simulink model "Mapping_cs"  (R2019a)
settings: Solver=ode5  StartTime=0.0  StopTime=inf  FixedStep=1/20  RelTol=1e-3
PreLoadFcn:
  | mbxruntime.callbacks.PreLoadFcn(bdroot);
PostLoadFcn:
  | mbxruntime.callbacks.PostLoadFcn(bdroot);
InitFcn:
  | mbxruntime.callbacks.InitFcn(bdroot);
StartFcn:
  | mbxruntime.callbacks.StartFcn(bdroot);
StopFcn:
  | mbxruntime.callbacks.StopFcn(bdroot);
model workspace: external: MAT-File .\Mapping_cs_hws.mat (data not in the file)
undefined symbols (not defined in the file or in its folder): InitImageOutputDir, Mapping_cs_BMW_X5_SUV_1_Path_pathUniqueID, Mapping_cs_BMW_X5_SUV_1_SpeedProfile_speedProfileUniqueID, mbxruntime
libraries: PreScanUsefulBlocks x1, adeye_lib x1
(part 1 of 2)
CloseFcn:
  | mbxruntime.callbacks.CloseFcn(bdroot);
settings Model: Creator=PRESCAN  LastModifiedBy=adeye
settings DataIOCC: LimitDataPoints=on  SaveFormat=Array  SignalLoggingSaveFormat=ModelDataLogs  ReturnWorkspaceOutputs=off
settings OptimizationCC: DefaultParameterBehavior=Inlined  ExpressionDepthLimit=2147483647  InitFltsAndDblsToZero=on  LifeSpan=inf
settings DebuggingCC: SaveWithParameterizedLinksMsg=none  UnderspecifiedInitializationDetection=Classic  MergeDetectMultiDrivingBlocksExec=none  SignalResolutionControl=TryResolveAllWithWarning  MultiTaskDSMMsg=warning  MultiTaskCondExecSysMsg=none  FcnCallInpInsideContextMsg=warning  StateNameClashWarn=warning  SFUnexpectedBacktrackingDiag=warning  SFNoUnconditionalDefaultTransitionDiag=warning  SFExecutionAtInitializationDiag=none  ArithmeticOperatorsInVariantConditions=warning
settings HardwareCC: ProdBitPerPointer=32  ProdBitPerSizeT=32  ProdBitPerPtrDiffT=32  ProdLargestAtomicFloat=None  ProdIntDivRoundTo=Undefined  ProdEndianess=Unspecified  ProdWordSize=32  ProdHWDeviceType=32-bit Generic
settings ModelReferenceCC: UpdateModelReferenceTargets=IfOutOfDate  PropagateSignalLabelsOutOfModel=off
settings SFSimCC: SimUseLocalCustomCode=off  SimParseCustomCode=off
settings SFSimCC: SimCustomHeaderCode=|
  | #include "prescan.h"
  | #include "prescan_platform.h"
  | #include "prescan_aimsunturnindicatorsetter_data.h"
settings RTWCC: RTWUseLocalCustomCode=off
settings CodeAppCC: StateflowObjectComments=on
settings GRTTargetCC: TargetFcnLib=ansi_tfl_tmw.mat  TargetLangStandard=C89/C90 (ANSI)  GeneratePreprocessorConditionals=Disable all  CombineOutputUpdateFcns=off  GRTInterface=on
settings ConfigComp: CovMetricSettings=dw  CovHtmlReporting=on  CovSaveCumulativeToWorkspaceVar=on  CovSaveSingleToWorkspaceVar=on  CovExternalEMLEnable=off  CovSFcnEnable=off

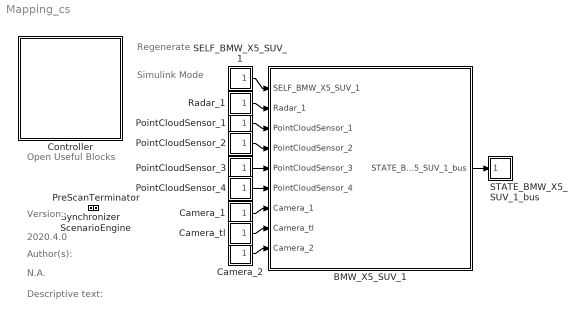
== system Mapping_cs ==
  note: Regenerate
  note: Simulink Mode
  note: Open Useful Blocks
  note: 2020.4.0
  note: Version:
  note: Author(s):
  note: N.A.
  note: Descriptive text:
  BMW_X5_SUV_1 : Subsystem  Tag=WorldObjectSubSystem  InitFcn=UniqueId = '158';
      mask init:
      | modelPath = GenericModelHelper.getGenericModelFilePath('ModelDepo','Vehicles\BMW_X5\BMW_X5.pgmb','bfeb1c11467705ab888b3011684c848b');imagePath = GenericModelHelper.getCompilationPicture(modelPath, 'BMW_X5_HighPoly.png');
      mask Display: image(imread(imagePath));color('white');text(0, 0, ' ID=10\n')
  Camera_1 : Subsystem  Tag=sensor/Camera/CameraSensor  Priority=30  mask(PreScan Source Block: Camera Sensor){}
      mask help: The Camera Sensor provides a color or monochrome image.
      settings: OpenFcn=open_system([gcb '/Sensor'],'mask')
      mask Help: eval('openHelp(457)')
      mask Display: image(imread('CameraSensor.png'))
  Camera_2 : Subsystem  Tag=sensor/Camera/CameraSensor  Priority=30  mask(PreScan Source Block: Camera Sensor){}
      mask help: The Camera Sensor provides a color or monochrome image.
      settings: OpenFcn=open_system([gcb '/Sensor'],'mask')
      mask Help: eval('openHelp(457)')
      mask Display: image(imread('CameraSensor.png'))
  Camera_tl : Subsystem  Tag=sensor/Camera/CameraSensor  Priority=30  mask(PreScan Source Block: Camera Sensor){}
      mask help: The Camera Sensor provides a color or monochrome image.
      settings: OpenFcn=open_system([gcb '/Sensor'],'mask')
      mask Help: eval('openHelp(457)')
      mask Display: image(imread('CameraSensor.png'))
  Controller : Subsystem  Description=8A3CD2955739A82C886C20AE3E253D78460D53180EE2C1B14CC08DF75A70BE77  Priority=-1  LoadFcn=load PreScanControllerData  mask(PreScan Simulation Controller){prescanversion='2020.4.0', ModelReferencing=off, TimeStep=1/20, ControlMode=0, PreScanExecutionMode=on, ControllerCount=0, ControllerIndex=0, ControllerOptions=''}
      mask prompts: prescanversion "PreScan Version"; ModelReferencing "Use Model Referencing"; TimeStep "Upload Period [s]"; ControlMode "Control Mode"; PreScanExecutionMode "Execution Mode"; ControllerCount "Controller Count"; ControllerIndex "Controller Index"; ControllerOptions "Controller Options"
      mask help:
      | Please do not remove this block from the compilation sheet,
      | as it connects the model to the PreScan environment.
      mask init:
      | model = bdroot(gcb);
      | ExperimentFile = mbxruntime.findExperimentFile(model,true); %relative path
      | 
      | [d1, d2, d3, prescandata] = prescan_Settings();
      | ModelDepo = fullfile(prescandata,'ModelDepo'); 
      | 
      | RTmode = mbxruntime.getRTMode(model);
      | 
      | SimulationMode = get_param(bdroot,'SimulationMode');
      | if strcmp(SimulationMode, 'rapid-accelerator')
      |     SimulationMode = 'external';
      | end
      | TargetName = get_param(bdroot,'SystemTargetFile');
      settings: ModelCloseFcn=assignin('base',['model_closed_' bdroot],true);
      mask Help: eval('openHelp(812)')
      mask Display: image(imread('prescanlogo.ico'))
  PointCloudSensor_1 : Subsystem  Tag=sensor/PointCloudInport  Priority=30  mask(PreScan Source Block: Point Cloud Sensor){}
      mask help: The Point Cloud Sensor provides XYZ positions relative to the sensor
      settings: OpenFcn=open_system([gcb '/Sensor'],'mask')
      mask Help: eval('openHelp(6400)')
      mask Display: image(imread('PointCloudSensorSL.png'))
  PointCloudSensor_2 : Subsystem  Tag=sensor/PointCloudInport  Priority=30  mask(PreScan Source Block: Point Cloud Sensor){}
      mask help: The Point Cloud Sensor provides XYZ positions relative to the sensor
      settings: OpenFcn=open_system([gcb '/Sensor'],'mask')
      mask Help: eval('openHelp(6400)')
      mask Display: image(imread('PointCloudSensorSL.png'))
  PointCloudSensor_3 : Subsystem  Tag=sensor/PointCloudInport  Priority=30  mask(PreScan Source Block: Point Cloud Sensor){}
      mask help: The Point Cloud Sensor provides XYZ positions relative to the sensor
      settings: OpenFcn=open_system([gcb '/Sensor'],'mask')
      mask Help: eval('openHelp(6400)')
      mask Display: image(imread('PointCloudSensorSL.png'))
  PointCloudSensor_4 : Subsystem  Tag=sensor/PointCloudInport  Priority=30  mask(PreScan Source Block: Point Cloud Sensor){}
      mask help: The Point Cloud Sensor provides XYZ positions relative to the sensor
      settings: OpenFcn=open_system([gcb '/Sensor'],'mask')
      mask Help: eval('openHelp(6400)')
      mask Display: image(imread('PointCloudSensorSL.png'))
  PreScanTerminator : Subsystem  Tag=PreScanTerminator  Priority=999  LoadFcn=load PrescanTerminatorData  mask(PreScan Simulation Terminator){TimeStep=1/20}
      mask prompts: TimeStep "Upload Period [s]"
      mask help:
      | Please do not remove this block from the compilation sheet as it
      | connects the model to the PreScan environment.
      mask Help: eval('openHelp(812)')
      mask Display: image(imread('prescanlogo.ico'))
  Radar_1 : Subsystem  Tag=sensor/Radar  Priority=30  LoadFcn=load('PrescanScannerSensorData.mat');load('PrescanScannerSensorMessage.mat')  mask(PreScan Source Block: Radar Sensor){}
      mask help:
      | The Radar Sensor is a detailed sensor based on a physical radar
      | model that includes Antenna GAIN Maps (AGM) and atmospheric
      | attenuation.
      |
      | For more information, please click Help.
      settings: OpenFcn=open_system([gcb '/Sensor'],'mask')
      mask Help: eval('openHelp(1464)')
      mask Display: image(imread('Radar.png'))
  SELF_BMW_X5_SUV_1 : Subsystem  Tag=sensor/SelfPort  Priority=30  LoadFcn=load('PreScanSelfSensorData.mat')  mask(PreScan Source Block: SELF){}
      mask help:
      | The SELF port shows (state) information of the actor itself. The outputs are position in the experiment's axis system and the GPS coordinates, and the object's absolute velocity and compass heading.
      |
      | For more information, please click Help.
      settings: OpenFcn=open_system([gcb '/Sensor'],'mask')
      mask Help: eval('openHelp(462)')
      mask Display: image(imread('GPS.png'))
  STATE_BMW_X5_SUV_1_bus : Subsystem  Tag=actuator/StatePort  Priority=0  LoadFcn=load('PreScanStateActuatorData.mat')  mask(PreScan Sink Block: State){}
      mask help:
      | The Actor State contains a vector signal of size (9x1), containing the following signals:
      |
      | -  Position    	(x,y,z)             	[m]
      | -  Velocity    	(vx,vy,vz)         	[m/s]
      | -  Angles       	(Roll, Pitch, Yaw)	[rad]
      |
      | The Actor state is defined in the global axis system.
      | The state is superponed on the Initial position defined in the GUI.
      |
      | For more information, please click Help.
      settings: OpenFcn=open_system([gcb '/Actuator'],'mask')
      mask Help: eval('openHelp(222)')
      mask Display: image(imread('State.png'))
  ScenarioEngine : Subsystem  Tag=PreScanOpenScenarioBlock  Priority=10  LoadFcn=load PrescanSynchronizeData  mask(PreScan Simulation Core Block){TimeStep=1/20}
      mask prompts: TimeStep "Timestep [s]"
      mask help:
      | Please do not remove this block from the PreScan compilation sheet,
      | as it contains essential configuration parameters for a PreScan simulation.
      settings: DeleteFcn=PreScanBlockDeleteFcn;
      mask Display: image(imread('prescanlogo.ico'))
  Synchronizer : Subsystem  Tag=PreScanSynchronizer  Priority=20  LoadFcn=load PrescanSynchronizeData  mask(PreScan Simulation Core Block){TimeStep=1/20}
      mask prompts: TimeStep "Timestep [s]"
      mask help:
      | Please do not remove this block from the PreScan compilation sheet,
      | as it contains essential configuration parameters for a PreScan simulation.
      settings: DeleteFcn=PreScanBlockDeleteFcn;
      mask Display: image(imread('prescanlogo.ico'))
  wires:
  BMW_X5_SUV_1/1(STATE_BMW_X5_SUV_1_bus) -> STATE_BMW_X5_SUV_1_bus/1(STATE_BMW_X5_SUV_1_bus)
  SELF_BMW_X5_SUV_1/1(SELF_BMW_X5_SUV_1) -> BMW_X5_SUV_1/1(SELF_BMW_X5_SUV_1)
  Radar_1/1(Radar_1) -> BMW_X5_SUV_1/2(Radar_1)
  PointCloudSensor_1/1(PointCloudSensor_1) -> BMW_X5_SUV_1/3(PointCloudSensor_1)
  PointCloudSensor_2/1(PointCloudSensor_2) -> BMW_X5_SUV_1/4(PointCloudSensor_2)
  PointCloudSensor_3/1(PointCloudSensor_3) -> BMW_X5_SUV_1/5(PointCloudSensor_3)
  PointCloudSensor_4/1(PointCloudSensor_4) -> BMW_X5_SUV_1/6(PointCloudSensor_4)
  Camera_1/1(Camera_1) -> BMW_X5_SUV_1/7(Camera_1)
  Camera_tl/1(Camera_tl) -> BMW_X5_SUV_1/8(Camera_tl)
  Camera_2/1(Camera_2) -> BMW_X5_SUV_1/9(Camera_2)

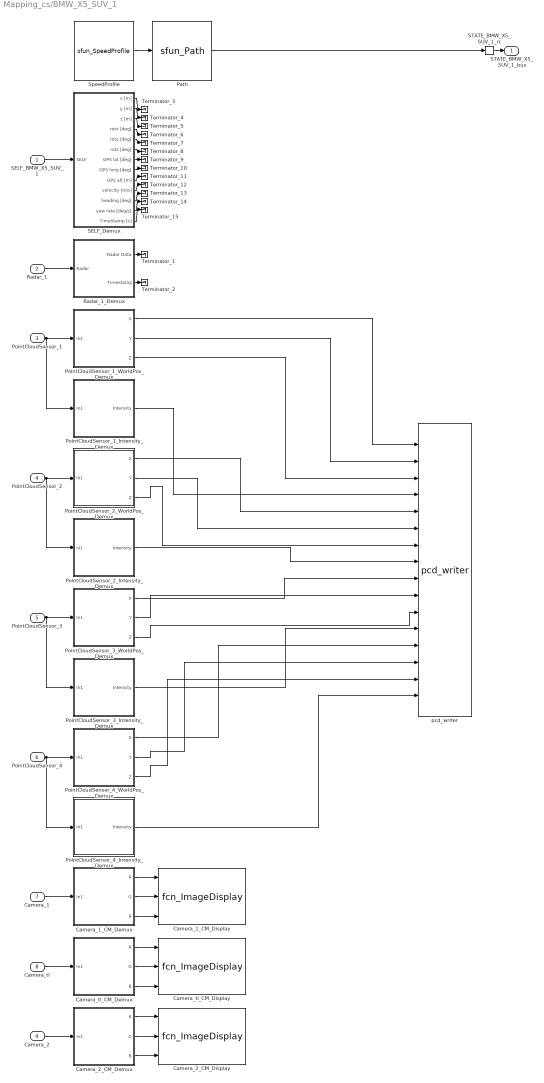
== system Mapping_cs/BMW_X5_SUV_1 ==
  SELF_BMW_X5_SUV_1 : Inport  Tag=inport/SelfPort  OutDataTypeStr=Bus: PRESCAN_SELFSENSORDATA  PortDimensions=1  SampleTime=1/20  BusOutputAsStruct=on
  Radar_1 : Inport  Tag=inport/Radar  Port=2  OutDataTypeStr=Bus: PRESCAN_SCANNERSENSOR_MESSAGE  PortDimensions=7  SampleTime=1/20  BusOutputAsStruct=on
  PointCloudSensor_1 : Inport  Tag=inport/PointCloudInport  Port=3  OutDataTypeStr=single  SampleTime=1/20  BusOutputAsStruct=on
  PointCloudSensor_2 : Inport  Tag=inport/PointCloudInport  Port=4  OutDataTypeStr=single  SampleTime=1/20  BusOutputAsStruct=on
  PointCloudSensor_3 : Inport  Tag=inport/PointCloudInport  Port=5  OutDataTypeStr=single  SampleTime=1/20  BusOutputAsStruct=on
  PointCloudSensor_4 : Inport  Tag=inport/PointCloudInport  Port=6  OutDataTypeStr=single  SampleTime=1/20  BusOutputAsStruct=on
  Camera_1 : Inport  Tag=inport/Camera/CameraSensor  Port=7  OutDataTypeStr=uint8  SampleTime=1/20  BusOutputAsStruct=on
  Camera_tl : Inport  Tag=inport/Camera/CameraSensor  Port=8  OutDataTypeStr=uint8  SampleTime=1/20  BusOutputAsStruct=on
  Camera_2 : Inport  Tag=inport/Camera/CameraSensor  Port=9  OutDataTypeStr=uint8  SampleTime=1/20  BusOutputAsStruct=on
  Camera_1_CM_Demux : Subsystem  Tag=demux/Camera/Color  mask{SensorName=Camera_1, hres=960, vres=720}
      mask prompts: SensorName "Sensor Name"; hres "Horizontal Resolution"; vres "Vertical Resolution"
      mask Help: eval('openHelp(457)')
      mask Display:
      | fprintf('MONO CAMERA:\n Color\n %s \n %d x %d px',SensorName,hres,vres)
      | port_label('output',1,'R')
      | port_label('output',2,'G')
      | port_label('output',3,'B')
  Camera_1_CM_Display : M-S-Function  Tag=CameraSensor_Color_Display  InitFcn=InitImageOutputDir(gcb);  FunctionName=fcn_ImageDisplay  Parameters=SensorName EnableDisplay EnablePosition DisplayPosition FigureHandle SaveResults BitmapFormat TempOutputDir CameraType DataType  mask(PreScan Color Display Block){SensorName=Camera_1, EnableDisplay=on, EnablePosition=off, DisplayPosition=[10 10 960 720], FigureHandle=15805, SaveResults=off, Format=PNG, TempOutputDir=0, CameraType=Mono, DataType=uint8}
      mask prompts: SensorName "User Specified: Title of Display"; EnableDisplay "Active"; EnablePosition "Set Display window position"; DisplayPosition "Display window position [xpos ypos width height]"; FigureHandle "Unique Handle"; SaveResults "Save results"; TempOutputDir "OutputDir"; CameraType "Camera Type"; DataType "Image Data Type"
      mask help: This block displays the RGB output of a PreScan camera sensor.
      mask init:
      | if EnableDisplay
      |     EnableString='';
      |     EnableColor='gray';
      | else
      |     EnableString='INACTIVE';
      |     EnableColor='red';
      | end
      | switch Format
      |     case 1
      |         BitmapFormat = 'png';
      |     case 2
      |         BitmapFormat = 'bmp';
      |     case 3
      |         BitmapFormat = 'jpg';
      | end 
      | if CameraType==1
      |     CameraTypeName='MONO';
      |     PortNumber=0;
      | else
      |     CameraTypeName='STEREO';
      |     PortNumber=3;
      | end
      settings: CopyFcn=CopyFcnDisplay  DeleteFcn=PreScanBlockDeleteFcn;  ModelCloseFcn=fcn_ImageDisplay_ModelCloseFcn
      mask Help: eval('openHelp(457)')
      mask Callback EnablePosition:
      | MV=get_param(gcb,'MaskVisibilities');
      | if strcmp(get_param(gcb,'EnablePosition'),'on')
      |     MV{4}='on';
      | else
      |     MV{4}='off';
      | end
      | set_param(gcb,'MaskVisibilities',MV);
      | clear MV;
      mask TypeOptions Format: PNG | BMP | JPG
      mask TypeOptions CameraType: Mono | Stereo
      mask TypeOptions DataType: uint8 | single
      mask Display:
      | color(EnableColor);
      | fprintf('%s\n DISPLAY:\n Color \n %s',EnableString,SensorName)
      | port_label('input',1,'R')
      | port_label('input',2,'G')
      | port_label('input',3,'B')
      | port_label('input',PortNumber+1,'R')
      | port_label('input',PortNumber+2,'G')
      | port_label('input',PortNumber+3,'B')
  Camera_2_CM_Demux : Subsystem  Tag=demux/Camera/Color  mask{SensorName=Camera_2, hres=960, vres=720}
      mask prompts: SensorName "Sensor Name"; hres "Horizontal Resolution"; vres "Vertical Resolution"
      mask Help: eval('openHelp(457)')
      mask Display:
      | fprintf('MONO CAMERA:\n Color\n %s \n %d x %d px',SensorName,hres,vres)
      | port_label('output',1,'R')
      | port_label('output',2,'G')
      | port_label('output',3,'B')
  Camera_2_CM_Display : M-S-Function  Tag=CameraSensor_Color_Display  InitFcn=InitImageOutputDir(gcb);  FunctionName=fcn_ImageDisplay  Parameters=SensorName EnableDisplay EnablePosition DisplayPosition FigureHandle SaveResults BitmapFormat TempOutputDir CameraType DataType  mask(PreScan Color Display Block){SensorName=Camera_2, EnableDisplay=on, EnablePosition=off, DisplayPosition=[10 10 960 720], FigureHandle=15807, SaveResults=off, Format=PNG, TempOutputDir=0, CameraType=Mono, DataType=uint8}
      mask prompts: SensorName "User Specified: Title of Display"; EnableDisplay "Active"; EnablePosition "Set Display window position"; DisplayPosition "Display window position [xpos ypos width height]"; FigureHandle "Unique Handle"; SaveResults "Save results"; TempOutputDir "OutputDir"; CameraType "Camera Type"; DataType "Image Data Type"
      mask help: This block displays the RGB output of a PreScan camera sensor.
      mask init: same as Mapping_cs/BMW_X5_SUV_1/Camera_1_CM_Display
      settings: CopyFcn=CopyFcnDisplay  DeleteFcn=PreScanBlockDeleteFcn;  ModelCloseFcn=fcn_ImageDisplay_ModelCloseFcn
      mask Help: eval('openHelp(457)')
      mask Callback EnablePosition:
      | MV=get_param(gcb,'MaskVisibilities');
      | if strcmp(get_param(gcb,'EnablePosition'),'on')
      |     MV{4}='on';
      | else
      |     MV{4}='off';
      | end
      | set_param(gcb,'MaskVisibilities',MV);
      | clear MV;
      mask TypeOptions Format: PNG | BMP | JPG
      mask TypeOptions CameraType: Mono | Stereo
      mask TypeOptions DataType: uint8 | single
      mask Display:
      | color(EnableColor);
      | fprintf('%s\n DISPLAY:\n Color \n %s',EnableString,SensorName)
      | port_label('input',1,'R')
      | port_label('input',2,'G')
      | port_label('input',3,'B')
      | port_label('input',PortNumber+1,'R')
      | port_label('input',PortNumber+2,'G')
      | port_label('input',PortNumber+3,'B')
  Camera_tl_CM_Demux : Subsystem  Tag=demux/Camera/Color  mask{SensorName=Camera_tl, hres=960, vres=720}
      mask prompts: SensorName "Sensor Name"; hres "Horizontal Resolution"; vres "Vertical Resolution"
      mask Help: eval('openHelp(457)')
      mask Display:
      | fprintf('MONO CAMERA:\n Color\n %s \n %d x %d px',SensorName,hres,vres)
      | port_label('output',1,'R')
      | port_label('output',2,'G')
      | port_label('output',3,'B')
  Camera_tl_CM_Display : M-S-Function  Tag=CameraSensor_Color_Display  InitFcn=InitImageOutputDir(gcb);  FunctionName=fcn_ImageDisplay  Parameters=SensorName EnableDisplay EnablePosition DisplayPosition FigureHandle SaveResults BitmapFormat TempOutputDir CameraType DataType  mask(PreScan Color Display Block){SensorName=Camera_tl, EnableDisplay=on, EnablePosition=off, DisplayPosition=[10 10 960 720], FigureHandle=15806, SaveResults=off, Format=PNG, TempOutputDir=0, CameraType=Mono, DataType=uint8}
      mask prompts: SensorName "User Specified: Title of Display"; EnableDisplay "Active"; EnablePosition "Set Display window position"; DisplayPosition "Display window position [xpos ypos width height]"; FigureHandle "Unique Handle"; SaveResults "Save results"; TempOutputDir "OutputDir"; CameraType "Camera Type"; DataType "Image Data Type"
      mask help: This block displays the RGB output of a PreScan camera sensor.
      mask init: same as Mapping_cs/BMW_X5_SUV_1/Camera_1_CM_Display
      settings: CopyFcn=CopyFcnDisplay  DeleteFcn=PreScanBlockDeleteFcn;  ModelCloseFcn=fcn_ImageDisplay_ModelCloseFcn
      mask Help: eval('openHelp(457)')
      mask Callback EnablePosition:
      | MV=get_param(gcb,'MaskVisibilities');
      | if strcmp(get_param(gcb,'EnablePosition'),'on')
      |     MV{4}='on';
      | else
      |     MV{4}='off';
      | end
      | set_param(gcb,'MaskVisibilities',MV);
      | clear MV;
      mask TypeOptions Format: PNG | BMP | JPG
      mask TypeOptions CameraType: Mono | Stereo
      mask TypeOptions DataType: uint8 | single
      mask Display:
      | color(EnableColor);
      | fprintf('%s\n DISPLAY:\n Color \n %s',EnableString,SensorName)
      | port_label('input',1,'R')
      | port_label('input',2,'G')
      | port_label('input',3,'B')
      | port_label('input',PortNumber+1,'R')
      | port_label('input',PortNumber+2,'G')
      | port_label('input',PortNumber+3,'B')
  Path : S-Function  LoadFcn=load('PrescanMotionData.mat')  FunctionName=sfun_Path  Parameters=mbxruntime.parameters.convert(uniqueID), pathUniqueID, mbxruntime.parameters.convert(timestep)  SFunctionDeploymentMode=off  EnableBusSupport=off  mask(Path){uniqueID=158, pathUniqueID=Mapping_cs_BMW_X5_SUV_1_Path_pathUniqueID, timestep=1/20}
      mask prompts: uniqueID "Object Unique ID"; pathUniqueID "Path Unique ID"; timestep "MATLAB timestep:"
      mask help:
      | The path block outputs the position along a given trajectory.
      |
      | For more information, please click Help.
      mask Help: eval('openHelp(312)')
      mask Display: image(imread('Path.png'))
  PointCloudSensor_1_Intensity_Demux : Subsystem  Tag=demux/PCS/Intensity  mask{SensorName=PointCloudSensor_1, offset=675, hres=225, vres=16}
      mask prompts: SensorName "Sensor Name"; offset "Data Start"; hres "Horizontal Resolution"; vres "Vertical Resolution"
      mask Help: eval('openHelp(6400)')
      mask Display:
      | fprintf('Point Cloud:\n Data\n %s \n %d x %d px',SensorName,hres,vres)
      | port_label('output',1,'Intensity')
  PointCloudSensor_1_WorldPos_Demux : Subsystem  Tag=demux/PCS/WorldPos  mask{SensorName=PointCloudSensor_1, offset=0, hres=225, vres=16}
      mask prompts: SensorName "Sensor Name"; offset "Data Start"; hres "Horizontal Resolution"; vres "Vertical Resolution"
      mask Help: eval('openHelp(6400)')
      mask Display:
      | fprintf('Point Cloud:\n Data\n %s \n %d x %d px',SensorName,hres,vres)
      | port_label('output',1,'X')
      | port_label('output',2,'Y')
      | port_label('output',3,'Z')
  PointCloudSensor_2_Intensity_Demux : Subsystem  Tag=demux/PCS/Intensity  mask{SensorName=PointCloudSensor_2, offset=675, hres=225, vres=16}
      mask prompts: SensorName "Sensor Name"; offset "Data Start"; hres "Horizontal Resolution"; vres "Vertical Resolution"
      mask Help: eval('openHelp(6400)')
      mask Display:
      | fprintf('Point Cloud:\n Data\n %s \n %d x %d px',SensorName,hres,vres)
      | port_label('output',1,'Intensity')
  PointCloudSensor_2_WorldPos_Demux : Subsystem  Tag=demux/PCS/WorldPos  mask{SensorName=PointCloudSensor_2, offset=0, hres=225, vres=16}
      mask prompts: SensorName "Sensor Name"; offset "Data Start"; hres "Horizontal Resolution"; vres "Vertical Resolution"
      mask Help: eval('openHelp(6400)')
      mask Display:
      | fprintf('Point Cloud:\n Data\n %s \n %d x %d px',SensorName,hres,vres)
      | port_label('output',1,'X')
      | port_label('output',2,'Y')
      | port_label('output',3,'Z')
  PointCloudSensor_3_Intensity_Demux : Subsystem  Tag=demux/PCS/Intensity  mask{SensorName=PointCloudSensor_3, offset=675, hres=225, vres=16}
      mask prompts: SensorName "Sensor Name"; offset "Data Start"; hres "Horizontal Resolution"; vres "Vertical Resolution"
      mask Help: eval('openHelp(6400)')
      mask Display:
      | fprintf('Point Cloud:\n Data\n %s \n %d x %d px',SensorName,hres,vres)
      | port_label('output',1,'Intensity')
  PointCloudSensor_3_WorldPos_Demux : Subsystem  Tag=demux/PCS/WorldPos  mask{SensorName=PointCloudSensor_3, offset=0, hres=225, vres=16}
      mask prompts: SensorName "Sensor Name"; offset "Data Start"; hres "Horizontal Resolution"; vres "Vertical Resolution"
      mask Help: eval('openHelp(6400)')
      mask Display:
      | fprintf('Point Cloud:\n Data\n %s \n %d x %d px',SensorName,hres,vres)
      | port_label('output',1,'X')
      | port_label('output',2,'Y')
      | port_label('output',3,'Z')
  PointCloudSensor_4_Intensity_Demux : Subsystem  Tag=demux/PCS/Intensity  mask{SensorName=PointCloudSensor_4, offset=675, hres=225, vres=16}
      mask prompts: SensorName "Sensor Name"; offset "Data Start"; hres "Horizontal Resolution"; vres "Vertical Resolution"
      mask Help: eval('openHelp(6400)')
      mask Display:
      | fprintf('Point Cloud:\n Data\n %s \n %d x %d px',SensorName,hres,vres)
      | port_label('output',1,'Intensity')
  PointCloudSensor_4_WorldPos_Demux : Subsystem  Tag=demux/PCS/WorldPos  mask{SensorName=PointCloudSensor_4, offset=0, hres=225, vres=16}
      mask prompts: SensorName "Sensor Name"; offset "Data Start"; hres "Horizontal Resolution"; vres "Vertical Resolution"
      mask Help: eval('openHelp(6400)')
      mask Display:
      | fprintf('Point Cloud:\n Data\n %s \n %d x %d px',SensorName,hres,vres)
      | port_label('output',1,'X')
      | port_label('output',2,'Y')
      | port_label('output',3,'Z')
  Radar_1_Demux : Subsystem  Tag=demux/Radar  TreatAsAtomicUnit=on  mask(PreScan Demux Block: Radar){MAXMESSAGES=7}
      mask prompts: MAXMESSAGES "Number of Objects"
      mask help:
      | The Radar Sensor is a detailed sensor based on a physical radar
      | model that includes Antenna GAIN Maps (AGM) and atmospheric
      | attenuation.
      |
      | For more information, please click Help.
      mask Help: eval('openHelp(1464)')
      mask Display:
      | port_label('input',1,'Radar')
      | port_label('output',1,'Radar Data')
      | port_label('output',2,'Timestamp [s]')
  SELF_Demux : Subsystem  Tag=demux/SelfPort  mask(PreScan Demux Block:){}
      mask help:
      | The SELF port shows (state) information of the actor itself. The outputs are position in the experiment's axis system and the GPS coordinates, and the object's absolute velocity and compass heading.
      |
      | For more information, please click Help.
      settings: DeleteFcn=PreScanBlockDeleteFcn;
      mask Help: eval('openHelp(462)')
      mask Display:
      | port_label('output',1,'x [m]')
      | port_label('output',2,'y [m]')
      | port_label('output',3,'z [m]','texmode','on')
      | port_label('output',4,'Rotx [deg]','texmode','on')
      | port_label('output',5,'Roty [deg]','texmode','on')
      | port_label('output',6,'Rotz [deg]','texmode','on')
      | port_label('output',7,'GPS lat [deg]','texmode','on')
      | port_label('output',8,'GPS long [deg]','texmode','on')
      | port_label('output',9,'GPS alt [m]','texmode','on')
      | port_label('output',10,'Velocity [m/s]')
      | port_label('output',11,'Heading [deg]')
      | port_label('output',12,'Yaw rate [deg/s]')
      | port_label('output',13,'Timestamp [s]')
  STATE_BMW_X5_SUV_1_rc : RateTransition  Tag=mux_rc/StatePort  OutPortSampleTimeOpt=Inherit
  SpeedProfile : S-Function  LoadFcn=load('PrescanMotionData.mat')  FunctionName=sfun_SpeedProfile  Parameters=speedProfileUniqueID, mbxruntime.parameters.convert(timestep)  SFunctionDeploymentMode=off  EnableBusSupport=off  mask(SpeedProfile){speedProfileUniqueID=Mapping_cs_BMW_X5_SUV_1_SpeedProfile_speedProfileUniqueID, timestep=1/20}
      mask prompts: speedProfileUniqueID "Speed Profile Unique ID"; timestep "MATLAB timestep:"
      mask help:
      | The speed profile block outputs the travelled distance, velocities and acceleration along a given path.
      |
      | For more information, please click Help.
      mask Help: eval('openHelp(312)')
      mask Display: image(imread('SpeedProfile.png'))
  Terminator_{1..15} (15 alike) : Terminator
  pcd_writer : adeye_lib/pcd_writer  SystemSampleTime=-1
  STATE_BMW_X5_SUV_1_bus : Outport  Tag=outport/StatePort  OutDataTypeStr=Bus: PRESCAN_STATEACTUATORDATA  PortDimensions=1  SampleTime=1/20
  wires:
  STATE_BMW_X5_SUV_1_rc/1 -> STATE_BMW_X5_SUV_1_bus/1
  SpeedProfile/1 -> Path/1
  Path/1 -> STATE_BMW_X5_SUV_1_rc/1
  SELF_BMW_X5_SUV_1/1 -> SELF_Demux/1(SELF)
  Radar_1/1 -> Radar_1_Demux/1(Radar)
  PointCloudSensor_1/1 -> PointCloudSensor_1_WorldPos_Demux/1(In1), PointCloudSensor_1_Intensity_Demux/1(In1)
  PointCloudSensor_1_WorldPos_Demux/1(X) -> pcd_writer/1
  PointCloudSensor_1_WorldPos_Demux/2(Y) -> pcd_writer/2
  PointCloudSensor_1_WorldPos_Demux/3(Z) -> pcd_writer/3
  PointCloudSensor_1_Intensity_Demux/1(Intensity) -> pcd_writer/4
  PointCloudSensor_2/1 -> PointCloudSensor_2_WorldPos_Demux/1(In1), PointCloudSensor_2_Intensity_Demux/1(In1)
  PointCloudSensor_2_WorldPos_Demux/1(X) -> pcd_writer/5
  PointCloudSensor_2_WorldPos_Demux/2(Y) -> pcd_writer/6
  PointCloudSensor_2_WorldPos_Demux/3(Z) -> pcd_writer/7
  PointCloudSensor_2_Intensity_Demux/1(Intensity) -> pcd_writer/8
  PointCloudSensor_3/1 -> PointCloudSensor_3_WorldPos_Demux/1(In1), PointCloudSensor_3_Intensity_Demux/1(In1)
  PointCloudSensor_3_WorldPos_Demux/1(X) -> pcd_writer/9
  PointCloudSensor_3_WorldPos_Demux/2(Y) -> pcd_writer/10
  PointCloudSensor_3_WorldPos_Demux/3(Z) -> pcd_writer/11
  PointCloudSensor_3_Intensity_Demux/1(Intensity) -> pcd_writer/12
  PointCloudSensor_4/1 -> PointCloudSensor_4_WorldPos_Demux/1(In1), PointCloudSensor_4_Intensity_Demux/1(In1)
  PointCloudSensor_4_WorldPos_Demux/1(X) -> pcd_writer/13
  PointCloudSensor_4_WorldPos_Demux/2(Y) -> pcd_writer/14
  PointCloudSensor_4_WorldPos_Demux/3(Z) -> pcd_writer/15
  PointCloudSensor_4_Intensity_Demux/1(Intensity) -> pcd_writer/16
  Camera_1/1 -> Camera_1_CM_Demux/1(In1)
  Camera_1_CM_Demux/1(R) -> Camera_1_CM_Display/1
  Camera_1_CM_Demux/2(G) -> Camera_1_CM_Display/2
  Camera_1_CM_Demux/3(B) -> Camera_1_CM_Display/3
  Camera_tl/1 -> Camera_tl_CM_Demux/1(In1)
  Camera_tl_CM_Demux/1(R) -> Camera_tl_CM_Display/1
  Camera_tl_CM_Demux/2(G) -> Camera_tl_CM_Display/2
  Camera_tl_CM_Demux/3(B) -> Camera_tl_CM_Display/3
  Camera_2/1 -> Camera_2_CM_Demux/1(In1)
  Camera_2_CM_Demux/1(R) -> Camera_2_CM_Display/1
  Camera_2_CM_Demux/2(G) -> Camera_2_CM_Display/2
  Camera_2_CM_Demux/3(B) -> Camera_2_CM_Display/3
  Radar_1_Demux/1(Radar Data) -> Terminator_1/1
  Radar_1_Demux/2(Timestamp) -> Terminator_2/1
  SELF_Demux/1(x [m]) -> Terminator_3/1
  SELF_Demux/2(y [m]) -> Terminator_4/1
  SELF_Demux/3(z [m]) -> Terminator_5/1
  SELF_Demux/4(rotx [deg]) -> Terminator_6/1
  SELF_Demux/5(roty [deg]) -> Terminator_7/1
  SELF_Demux/6(rotz [deg]) -> Terminator_8/1
  SELF_Demux/7(GPS lat [deg]) -> Terminator_9/1
  SELF_Demux/8(GPS long [deg]) -> Terminator_10/1
  SELF_Demux/9(GPS alt [m]) -> Terminator_11/1
  SELF_Demux/10(velocity [m/s]) -> Terminator_12/1
  SELF_Demux/11(heading [deg]) -> Terminator_13/1
  SELF_Demux/12(yaw rate [deg/s]) -> Terminator_14/1
  SELF_Demux/13(TimeStamp [s]) -> Terminator_15/1

== system Mapping_cs/Camera_1 ==
  Sensor : S-Function  FunctionName=sfun_Camera  Parameters=mbxruntime.parameters.convert(sensorID), mbxruntime.parameters.convert(dataWidth), mbxruntime.parameters.convert(dataHeight), mbxruntime.parameters.convert(channelsPerImage), mbxruntime.parameters.convert(numberOfImages), mbxruntime.parameters.convert(timestep)  SFunctionDeploymentMode=off  EnableBusSupport=off  mask(PreScan Source Block: Camera Sensor){sensorID=163, dataWidth=720, dataHeight=2880, channelsPerImage=3, numberOfImages=1, timestep=1/20}
      mask prompts: sensorID "Sensor ID"; dataWidth "Data width"; dataHeight "Data Height"; channelsPerImage "Channels per image"; numberOfImages "Number of images"; timestep "MATLAB timestep:"
      mask help: The Camera Sensor provides a color or monochrome image.
      mask Help: eval('openHelp(457)')
      mask Display: image(imread('CameraSensor.png'))
  Camera_1 : Outport  Tag=outport/Camera/CameraSensor  OutDataTypeStr=uint8  SampleTime=1/20
  wires:
  Sensor/1 -> Camera_1/1

== system Mapping_cs/Camera_2 ==
  Sensor : S-Function  FunctionName=sfun_Camera  Parameters=mbxruntime.parameters.convert(sensorID), mbxruntime.parameters.convert(dataWidth), mbxruntime.parameters.convert(dataHeight), mbxruntime.parameters.convert(channelsPerImage), mbxruntime.parameters.convert(numberOfImages), mbxruntime.parameters.convert(timestep)  SFunctionDeploymentMode=off  EnableBusSupport=off  mask(PreScan Source Block: Camera Sensor){sensorID=166, dataWidth=720, dataHeight=2880, channelsPerImage=3, numberOfImages=1, timestep=1/20}
      mask prompts: sensorID "Sensor ID"; dataWidth "Data width"; dataHeight "Data Height"; channelsPerImage "Channels per image"; numberOfImages "Number of images"; timestep "MATLAB timestep:"
      mask help: The Camera Sensor provides a color or monochrome image.
      mask Help: eval('openHelp(457)')
      mask Display: image(imread('CameraSensor.png'))
  Camera_2 : Outport  Tag=outport/Camera/CameraSensor  OutDataTypeStr=uint8  SampleTime=1/20
  wires:
  Sensor/1 -> Camera_2/1

== system Mapping_cs/Camera_tl ==
  Sensor : S-Function  FunctionName=sfun_Camera  Parameters=mbxruntime.parameters.convert(sensorID), mbxruntime.parameters.convert(dataWidth), mbxruntime.parameters.convert(dataHeight), mbxruntime.parameters.convert(channelsPerImage), mbxruntime.parameters.convert(numberOfImages), mbxruntime.parameters.convert(timestep)  SFunctionDeploymentMode=off  EnableBusSupport=off  mask(PreScan Source Block: Camera Sensor){sensorID=164, dataWidth=720, dataHeight=2880, channelsPerImage=3, numberOfImages=1, timestep=1/20}
      mask prompts: sensorID "Sensor ID"; dataWidth "Data width"; dataHeight "Data Height"; channelsPerImage "Channels per image"; numberOfImages "Number of images"; timestep "MATLAB timestep:"
      mask help: The Camera Sensor provides a color or monochrome image.
      mask Help: eval('openHelp(457)')
      mask Display: image(imread('CameraSensor.png'))
  Camera_tl : Outport  Tag=outport/Camera/CameraSensor  OutDataTypeStr=uint8  SampleTime=1/20
  wires:
  Sensor/1 -> Camera_tl/1

== system Mapping_cs/Controller ==
  Terminator : Terminator
  sfun_Controller : S-Function  FunctionName=sfun_Controller  Parameters=SParameter1, SParameter2, SParameter3, SParameter4, SParameter5, SParameter6, SParameter7, SParameter8, SParameter9, SParameter10, SampleTime  SFunctionDeploymentMode=off  EnableBusSupport=off  mask(Legacy Function){SFunctionSpec=void prescan_outputFcn(void** work1, PRESCAN_CONTROLLERDATA y1[1]), SParameter1=uint8([ExperimentFile 0]), SParameter2=uint8([ModelDepo 0]), SParameter3=uint8([ControllerOptions 0]), SParameter4=RTmode, SParameter5=PreScanExecutionMode, SParameter6=ControlMode, SParameter7=ControllerCount, SParameter8=ControllerIndex, SParameter9=uint8([SimulationMode 0]), SParameter10=uint8([TargetName 0]), SampleTime=TimeStep, ShowSpec=on}
      mask prompts: SParameter1 "P1:"; SParameter2 "P2:"; SParameter3 "P3:"; SParameter4 "P4:"; SParameter5 "P5:"; SParameter6 "P6:"; SParameter7 "P7:"; SParameter8 "P8:"; SParameter9 "P9:"; SParameter10 "P10:"; SampleTime "Sample time (-1 for inherited):"; ShowSpec "Display function specification"
      mask help:
      | This block allows you to call the legacy functions specified by the following Legacy Code Tool definition:
      | def.SFunctionName = 'sfun_Controller';
      | def.OutputFcnSpec = 'void prescan_outputFcn(void** work1, PRESCAN_CONTROLLERDATA y1[1])';
      | def.StartFcnSpec = 'void prescan_startFcn(void ** work1, uint8 p1[], uint8 p2[], uint8 p3[], double p4, double p5, double p6, double p7, double p8, uint8 p9[], uint8 p10[])';
      | def.TerminateFcnSpec = 'void prescan_terminateFcn(void** work1)';
      | def.HeaderFiles = {'prescan_controller_data.h', 'prescan_SFunLibrary.h', 'prescan_CreateLogHandler.h', 'prescan_CreateErrorHandler.h', 'prescan_modify.h', 'ModuleDLL.h'};
      | def.SourceFiles = {'prescan_MexLogHandler.c', 'prescan_SimStructErrorHandler.c', 'prescan_LogHandler.c', 'prescan_ErrorHandler.c', 'prescan_Modify.c'};
      | def.HostLibFiles = {'sensorinterfaced.lib'};
      | def.TargetLibFiles = {'sensorinterfaced.so'};
      | def.IncPaths = {'.', 'C:\projects\prescan\rt_vislibrary\vis\..\pimp\include\sensors\InterfaceRTW'};
      | def.SrcPaths = {'C:\projects\prescan\rt_vislibrary\vis\..\pimp\include\sensors\InterfaceRTW', 'C:\projects\prescan\rt_vislibrary\vis\..\pimp\include\sensors\InterfaceRTW\ccurrt'};
      | def.LibPaths = {'C:\\projects\\prescan\\vislibrary_build\lib'};
      | def.SampleTime = 'parameterized';
      mask Help: <p>This block was generated automatically by the Legacy Code Tool. For detailed help on this tool, call<a href="matlab:legacy_code('help')"> legacy_code('help')</a>.</p>
      mask Callback ShowSpec:
      | if strcmp(get_param(gcbh, 'ShowSpec'), 'on')
      |   set_param(gcbh, 'MaskDisplay', sprintf('fprintf(''%s'');', get_param(gcbh, 'SFunctionSpec')));
      | else
      |   set_param(gcbh, 'MaskDisplay', sprintf('fprintf(''%s'');', get_param(gcbh, 'FunctionName')));
      | end
      mask Display: fprintf('void prescan_outputFcn(void** work1, PRESCAN_CONTROLLERDATA y1[1])');
  wires:
  sfun_Controller/1 -> Terminator/1

== system Mapping_cs/PointCloudSensor_1 ==
  Sensor : S-Function  FunctionName=sfun_PCS  Parameters=mbxruntime.parameters.convert(sensorID), mbxruntime.parameters.convert(dataWidth), mbxruntime.parameters.convert(dataHeight), mbxruntime.parameters.convert(numChannels), mbxruntime.parameters.convert(dataType), mbxruntime.parameters.convert(timestep)  SFunctionDeploymentMode=off  EnableBusSupport=off  mask(PreScan Source Block: Point Cloud Sensor){sensorID=159, dataWidth=16, dataHeight=900, numChannels=4, dataType=0, timestep=1/20}
      mask prompts: sensorID "Sensor ID"; dataWidth "Data Width"; dataHeight "Data Height"; numChannels "Channel Count"; dataType "Data Type"; timestep "MATLAB timestep:"
      mask help: The Point Cloud Sensor provides XYZ positions relative to the sensor
      mask Help: eval('openHelp(6400)')
      mask Display: image(imread('PointCloudSensorSL.png'))
  PointCloudSensor_1 : Outport  Tag=outport/PointCloudInport  OutDataTypeStr=single  SampleTime=1/20
  wires:
  Sensor/1 -> PointCloudSensor_1/1

== system Mapping_cs/PointCloudSensor_2 ==
  Sensor : S-Function  FunctionName=sfun_PCS  Parameters=mbxruntime.parameters.convert(sensorID), mbxruntime.parameters.convert(dataWidth), mbxruntime.parameters.convert(dataHeight), mbxruntime.parameters.convert(numChannels), mbxruntime.parameters.convert(dataType), mbxruntime.parameters.convert(timestep)  SFunctionDeploymentMode=off  EnableBusSupport=off  mask(PreScan Source Block: Point Cloud Sensor){sensorID=160, dataWidth=16, dataHeight=900, numChannels=4, dataType=0, timestep=1/20}
      mask prompts: sensorID "Sensor ID"; dataWidth "Data Width"; dataHeight "Data Height"; numChannels "Channel Count"; dataType "Data Type"; timestep "MATLAB timestep:"
      mask help: The Point Cloud Sensor provides XYZ positions relative to the sensor
      mask Help: eval('openHelp(6400)')
      mask Display: image(imread('PointCloudSensorSL.png'))
  PointCloudSensor_2 : Outport  Tag=outport/PointCloudInport  OutDataTypeStr=single  SampleTime=1/20
  wires:
  Sensor/1 -> PointCloudSensor_2/1

== system Mapping_cs/PointCloudSensor_3 ==
  Sensor : S-Function  FunctionName=sfun_PCS  Parameters=mbxruntime.parameters.convert(sensorID), mbxruntime.parameters.convert(dataWidth), mbxruntime.parameters.convert(dataHeight), mbxruntime.parameters.convert(numChannels), mbxruntime.parameters.convert(dataType), mbxruntime.parameters.convert(timestep)  SFunctionDeploymentMode=off  EnableBusSupport=off  mask(PreScan Source Block: Point Cloud Sensor){sensorID=161, dataWidth=16, dataHeight=900, numChannels=4, dataType=0, timestep=1/20}
      mask prompts: sensorID "Sensor ID"; dataWidth "Data Width"; dataHeight "Data Height"; numChannels "Channel Count"; dataType "Data Type"; timestep "MATLAB timestep:"
      mask help: The Point Cloud Sensor provides XYZ positions relative to the sensor
      mask Help: eval('openHelp(6400)')
      mask Display: image(imread('PointCloudSensorSL.png'))
  PointCloudSensor_3 : Outport  Tag=outport/PointCloudInport  OutDataTypeStr=single  SampleTime=1/20
  wires:
  Sensor/1 -> PointCloudSensor_3/1

== system Mapping_cs/PointCloudSensor_4 ==
  Sensor : S-Function  FunctionName=sfun_PCS  Parameters=mbxruntime.parameters.convert(sensorID), mbxruntime.parameters.convert(dataWidth), mbxruntime.parameters.convert(dataHeight), mbxruntime.parameters.convert(numChannels), mbxruntime.parameters.convert(dataType), mbxruntime.parameters.convert(timestep)  SFunctionDeploymentMode=off  EnableBusSupport=off  mask(PreScan Source Block: Point Cloud Sensor){sensorID=162, dataWidth=16, dataHeight=900, numChannels=4, dataType=0, timestep=1/20}
      mask prompts: sensorID "Sensor ID"; dataWidth "Data Width"; dataHeight "Data Height"; numChannels "Channel Count"; dataType "Data Type"; timestep "MATLAB timestep:"
      mask help: The Point Cloud Sensor provides XYZ positions relative to the sensor
      mask Help: eval('openHelp(6400)')
      mask Display: image(imread('PointCloudSensorSL.png'))
  PointCloudSensor_4 : Outport  Tag=outport/PointCloudInport  OutDataTypeStr=single  SampleTime=1/20
  wires:
  Sensor/1 -> PointCloudSensor_4/1

== system Mapping_cs/PreScanTerminator ==
  Terminator : Terminator
  sfun_Terminator : S-Function  FunctionName=sfun_Terminator  Parameters=SampleTime  SFunctionDeploymentMode=off  EnableBusSupport=off  mask(Legacy Function){SFunctionSpec=void prescan_terminator_outputFcn(void ** work1, PRESCAN_TERMINATORDATA y1[1]), SampleTime=TimeStep, ShowSpec=on}
      mask prompts: SampleTime "Sample time (-1 for inherited):"; ShowSpec "Display function specification"
      mask help:
      | This block allows you to call the legacy functions specified by the following Legacy Code Tool definition:
      | def.SFunctionName = 'sfun_Terminator';
      | def.OutputFcnSpec = 'void prescan_terminator_outputFcn(void ** work1, PRESCAN_TERMINATORDATA y1[1])';
      | def.StartFcnSpec = 'void prescan_terminator_startFcn(void ** work1)';
      | def.TerminateFcnSpec = 'void prescan_terminator_terminateFcn(void ** work1)';
      | def.HeaderFiles = {'prescan_terminator_data.h'};
      | def.HostLibFiles = {'sensorinterfaced.lib'};
      | def.IncPaths = {'src', 'C:\prescandev\vislibrary\vis\..\pimp\include\sensors\InterfaceRTW'};
      | def.SrcPaths = {'src'};
      | def.LibPaths = {'C:\\prescandev\\vislibrary_build\lib'};
      | def.SampleTime = 'parameterized';
      | def.Options.language = 'C';
      mask Help: <p>This block was generated automatically by the Legacy Code Tool. For detailed help on this tool, call<a href="matlab:legacy_code('help')"> legacy_code('help')</a>.</p>
      mask Callback ShowSpec:
      | if strcmp(get_param(gcbh, 'ShowSpec'), 'on')
      |   set_param(gcbh, 'MaskDisplay', sprintf('fprintf(''%s'');', get_param(gcbh, 'SFunctionSpec')));
      | else
      |   set_param(gcbh, 'MaskDisplay', sprintf('fprintf(''%s'');', get_param(gcbh, 'FunctionName')));
      | end
      mask Display: fprintf('void prescan_terminator_outputFcn(void ** work1, PRESCAN_TERMINATORDATA y1[1])');
  wires:
  sfun_Terminator/1 -> Terminator/1

== system Mapping_cs/Radar_1 ==
  Sensor : S-Function  FunctionName=sfun_Radar  Parameters=mbxruntime.parameters.convert(sensorID), mbxruntime.parameters.convert(detectableObjects), mbxruntime.parameters.convert(timestep)  SFunctionDeploymentMode=off  EnableBusSupport=off  mask(PreScan Source Block: Radar Sensor){sensorID=165, detectableObjects=7, timestep=1/20}
      mask prompts: sensorID "Sensor ID"; detectableObjects "Max detectable objects:"; timestep "MATLAB timestep:"
      mask help:
      | The Radar Sensor is a detailed sensor based on a physical radar
      | model that includes Antenna GAIN Maps (AGM) and atmospheric
      | attenuation.
      |
      | For more information, please click Help.
      mask Help: eval('openHelp(1464)')
      mask Display: image(imread('Radar.png'))
  Radar_1 : Outport  Tag=outport/Radar  OutDataTypeStr=Bus: PRESCAN_SCANNERSENSOR_MESSAGE  PortDimensions=7  SampleTime=1/20
  wires:
  Sensor/1 -> Radar_1/1

== system Mapping_cs/SELF_BMW_X5_SUV_1 ==
  Sensor : S-Function  FunctionName=sfun_SelfSensor  Parameters=mbxruntime.parameters.convert(UniqueID), mbxruntime.parameters.convert(TimeStep)  SFunctionDeploymentMode=off  EnableBusSupport=off  mask(PreScan Source Block: SELF){UniqueID=158, TimeStep=1/20}
      mask prompts: UniqueID "Auto-Assigned: Unique ID"; TimeStep "Auto-Assigned: Upload Period [s]"
      mask help:
      | The SELF port shows (state) information of the actor itself. The outputs are position in the experiment's axis system and the GPS coordinates, and the object's absolute velocity and compass heading.
      |
      | For more information, please click Help.
      mask Help: eval('openHelp(462)')
      mask Display: image(imread('GPS.png'))
  SELF_BMW_X5_SUV_1 : Outport  Tag=outport/SelfPort  OutDataTypeStr=Bus: PRESCAN_SELFSENSORDATA  PortDimensions=1  SampleTime=1/20
  wires:
  Sensor/1 -> SELF_BMW_X5_SUV_1/1

== system Mapping_cs/STATE_BMW_X5_SUV_1_bus ==
  STATE_BMW_X5_SUV_1_bus : Inport  Tag=inport/StatePort  OutDataTypeStr=Bus: PRESCAN_STATEACTUATORDATA  PortDimensions=1  SampleTime=1/20  BusOutputAsStruct=on
  Actuator : S-Function  FunctionName=sfun_StateActuator  Parameters=mbxruntime.parameters.convert(UniqueID), mbxruntime.parameters.convert(TimeStep)  SFunctionDeploymentMode=off  EnableBusSupport=off  mask(PreScan Sink Block: State){UniqueID=158, TimeStep=1/20}
      mask prompts: UniqueID "Auto-Assigned: Unique ID"; TimeStep "Auto-Assigned: Upload Period [s]"
      mask help:
      | The Actor State contains a vector signal of size (9x1), containing the following signals:
      |
      | -  Position    	(x,y,z)             	[m]
      | -  Velocity    	(vx,vy,vz)         	[m/s]
      | -  Angles       	(Roll, Pitch, Yaw)	[rad]
      |
      | The Actor state is defined in the global axis system.
      | The state is superponed on the Initial position defined in the GUI.
      |
      | For more information, please click Help.
      mask Help: eval('openHelp(222)')
      mask Display: image(imread('State.png'))
  wires:
  STATE_BMW_X5_SUV_1_bus/1 -> Actuator/1

== system Mapping_cs/ScenarioEngine ==
  Clock : Clock
  sfun_ScenarioEngine : S-Function  FunctionName=sfun_ScenarioEngine  Parameters=TimeStep  SFunctionDeploymentMode=off  EnableBusSupport=off
  wires:
  Clock/1 -> sfun_ScenarioEngine/1

== system Mapping_cs/Synchronizer ==
  Bus Selector1 : BusSelector  OutputSignals=FederateStopped
  Stop Simulation : Stop
  sfun_Synchronizer : S-Function  FunctionName=sfun_Synchronizer  Parameters=SampleTime  SFunctionDeploymentMode=off  EnableBusSupport=off  mask(Legacy Function){SFunctionSpec=void prescan_synchronizer_outputFcn(void ** work1, PRESCAN_SYNCHRONIZEDATA y1[1]), SampleTime=TimeStep, ShowSpec=on}
      mask prompts: SampleTime "Sample time (-1 for inherited):"; ShowSpec "Display function specification"
      mask help:
      | This block allows you to call the legacy functions specified by the following Legacy Code Tool definition:
      | def.SFunctionName = 'sfun_Synchronizer';
      | def.OutputFcnSpec = 'void prescan_synchronizer_outputFcn(void ** work1, PRESCAN_TIMESTAMPDATA u1[1], PRESCAN_SYNCHRONIZEDATA y1[1])';
      | def.StartFcnSpec = 'void prescan_synchronizer_startFcn(void ** work1)';
      | def.TerminateFcnSpec = 'void prescan_synchronizer_terminateFcn(void ** work1)';
      | def.HeaderFiles = {'prescan_synchronizer_data.h'};
      | def.HostLibFiles = {'sensorinterfaced.lib'};
      | def.IncPaths = {'src', 'C:\prescandev\vislibrary\vis\..\pimp\include\sensors\InterfaceRTW'};
      | def.SrcPaths = {'src'};
      | def.LibPaths = {'C:\\prescandev\\vislibrary_build\lib'};
      | def.SampleTime = 'parameterized';
      | def.Options.language = 'C';
      mask Help: <p>This block was generated automatically by the Legacy Code Tool. For detailed help on this tool, call<a href="matlab:legacy_code('help')"> legacy_code('help')</a>.</p>
      mask Callback ShowSpec:
      | if strcmp(get_param(gcbh, 'ShowSpec'), 'on')
      |   set_param(gcbh, 'MaskDisplay', sprintf('fprintf(''%s'');', get_param(gcbh, 'SFunctionSpec')));
      | else
      |   set_param(gcbh, 'MaskDisplay', sprintf('fprintf(''%s'');', get_param(gcbh, 'FunctionName')));
      | end
      mask Display: fprintf('void prescan_synchronizer_outputFcn(void ** work1, PRESCAN_SYNCHRONIZEDATA y1[1])');
  wires:
  sfun_Synchronizer/1 -> Bus Selector1/1
  Bus Selector1/1 -> Stop Simulation/1  "<FederateStopped>"

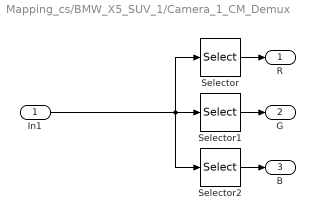
== system Mapping_cs/BMW_X5_SUV_1/Camera_1_CM_Demux ==
  In1 : Inport
  Selector : Selector  NumberOfDimensions=2  InputPortWidth=3  IndexOptions=Index vector (dialog),Index vector (dialog)  Indices=-1,1:hres  OutputSizes=1,1
  Selector1 : Selector  NumberOfDimensions=2  InputPortWidth=3  IndexOptions=Index vector (dialog),Index vector (dialog)  Indices=-1,hres+1:hres*2  OutputSizes=1,1
  Selector2 : Selector  NumberOfDimensions=2  InputPortWidth=3  IndexOptions=Index vector (dialog),Index vector (dialog)  Indices=-1,hres*2+1:hres*3  OutputSizes=1,1
  R : Outport
  G : Outport  Port=2
  B : Outport  Port=3
  wires:
  In1/1 -> Selector1/1, Selector/1, Selector2/1
  Selector/1 -> R/1
  Selector1/1 -> G/1
  Selector2/1 -> B/1

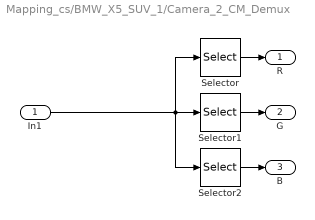
== system Mapping_cs/BMW_X5_SUV_1/Camera_2_CM_Demux ==
  In1 : Inport
  Selector : Selector  NumberOfDimensions=2  InputPortWidth=3  IndexOptions=Index vector (dialog),Index vector (dialog)  Indices=-1,1:hres  OutputSizes=1,1
  Selector1 : Selector  NumberOfDimensions=2  InputPortWidth=3  IndexOptions=Index vector (dialog),Index vector (dialog)  Indices=-1,hres+1:hres*2  OutputSizes=1,1
  Selector2 : Selector  NumberOfDimensions=2  InputPortWidth=3  IndexOptions=Index vector (dialog),Index vector (dialog)  Indices=-1,hres*2+1:hres*3  OutputSizes=1,1
  R : Outport
  G : Outport  Port=2
  B : Outport  Port=3
  wires:
  In1/1 -> Selector1/1, Selector/1, Selector2/1
  Selector/1 -> R/1
  Selector1/1 -> G/1
  Selector2/1 -> B/1

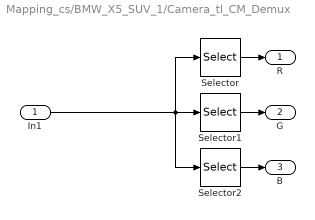
== system Mapping_cs/BMW_X5_SUV_1/Camera_tl_CM_Demux ==
  In1 : Inport
  Selector : Selector  NumberOfDimensions=2  InputPortWidth=3  IndexOptions=Index vector (dialog),Index vector (dialog)  Indices=-1,1:hres  OutputSizes=1,1
  Selector1 : Selector  NumberOfDimensions=2  InputPortWidth=3  IndexOptions=Index vector (dialog),Index vector (dialog)  Indices=-1,hres+1:hres*2  OutputSizes=1,1
  Selector2 : Selector  NumberOfDimensions=2  InputPortWidth=3  IndexOptions=Index vector (dialog),Index vector (dialog)  Indices=-1,hres*2+1:hres*3  OutputSizes=1,1
  R : Outport
  G : Outport  Port=2
  B : Outport  Port=3
  wires:
  In1/1 -> Selector1/1, Selector/1, Selector2/1
  Selector/1 -> R/1
  Selector1/1 -> G/1
  Selector2/1 -> B/1

== system Mapping_cs/BMW_X5_SUV_1/PointCloudSensor_1_Intensity_Demux ==
  In1 : Inport
  Selector3 : Selector  NumberOfDimensions=2  InputPortWidth=3  IndexOptions=Index vector (dialog),Index vector (dialog)  Indices=-1,offset+1:(offset+hres)  OutputSizes=1,1
  Intensity : Outport
  wires:
  Selector3/1 -> Intensity/1
  In1/1 -> Selector3/1
